simulink model "ZT_VehCtrl_18B_CAN"  (R2018b)
settings: Solver=FixedStepAuto  StartTime=0.0  StopTime=inf  FixedStep=0.005  RelTol=1e-3
InitFcn:
  | mbd_mpc_consistency_checks(bdroot(gcs));
values from neighbouring files (symbols this model uses):
  BatoverTempTh = single(80)    [VCU_INIT.m]
  BRS_PwrValid = single(5)    [VCU_INIT.m]
  BRSEnSpdTh1 = single(10)    [VCU_INIT.m]
  BRSEnSpdTh2 = single(20)    [VCU_INIT.m]
  MCUTempAlarmTh = single (60)    [VCU_INIT.m]
  mps2kmh = single(3.6)    [VCU_INIT.m]
  MtrPwrFac = single(1/9550)    [VCU_INIT.m]
  MtrTempAlarmTh = single (50)    [VCU_INIT.m]
  Padle1Signal1_Th = [PadleSignal1_min,PadleSignal1_max]    [VCU_INIT.m]
  Padle1Signal2_Th = [PadleSignal2_min,PadleSignal2_max]    [VCU_INIT.m]
  PadleSignal1_max = 3.84    [VCU_INIT.m]
  PadleSignal1_min = 0.75    [VCU_INIT.m]
  PadleSignal2_max = 1.92    [VCU_INIT.m]
  PadleSignal2_min = 0.375    [VCU_INIT.m]
  PadleValid = 0.05    [VCU_INIT.m]
  PwrLimFactor = single(0.5)    [VCU_INIT.m]
  Ratio = single(1)    [VCU_INIT.m]
  rpm2mps = single(2*pi/60 * WhlRadius/Ratio)    [VCU_INIT.m]
  SOCLowTh = single(20)    [VCU_INIT.m]
  VehPwrBackwardMax = VehPwrMax * single(0.3)    [VCU_INIT.m]
  VehPwrMax = single(MtrPwrMax * 4)    [VCU_INIT.m]
  VehTrqBackwardMax = VehTrqMax * single(0.3)    [VCU_INIT.m]
  VehTrqMax = single(MtrTrqMax * Ratio *4)    [VCU_INIT.m]
  WhlRadius = single(1)    [VCU_INIT.m]
undefined symbols (not defined in the file or in its folder): Delay_Charge, Delay_Discharge, fifo_0_vect, fifo_1_vect, LQFP, pts1_fifo_0_vect, pts1_fifo_1_vect, pts2_fifo_0_vect, pts2_fifo_1_vect, pts3_fifo_0_vect, pts3_fifo_1_vect, pts4_fifo_0_vect, pts4_fifo_1_vect
libraries: mbd_mpc574x_ec_toolbox x157, canmsglib x74, simulink x38
(part 9 of 12)

== system ZT_VehCtrl_18B_CAN/SigIn/CAN0 /BMS_Relay Status2/UNPACK ==
  ID : Inport
  data : Inport  Port=2
  length : Inport  Port=3
  timestamp : Inport  Port=4
  Action Port : ActionPort
  Bus Creator : BusCreator  Inputs=7  OutDataTypeStr=Bus: CAN_MESSAGE_BUS  NonVirtualBus=on
  Bus Creator1 : BusCreator  Inputs=2
  CAN Unpack6 : canmsglib/CAN Unpack  CANdbFile=D:\VCU\VCU_SL_ZhengZhou\ZT2\模型与接口\CAN_DBC\整车CANA_GBK.dbc  MsgList=(none)  MsgName=BMS_Relay_Status_2  MsgIDType=Standard (11-bit identifier)  MsgIdentifier=864  MsgLength=8  SignalInfo=NO1_RelayFaultStatus$9$2$2$2$1$0$1$0$0$3$#NO1_RelayIndex$11$5$2$2$1$0$1$0$0$31$#NO1_RelayStatus$8$1$2$2$1$0$1$0$0$1$#NO2_RelayFaultStatus$17$2$2$2$1$0$1$0$0$3$#NO2_RelayIndex$19$5$2$2$1$0$1$0$0$31$#NO2_RelayStatus$16$1$2$2$1$0$1$0$0$1$#NO3_RelayFaultStatus$25$2$2$2$1$0$1$0$0$3$#NO3_RelayIndex$27$5$2$2$1$0$1$0$0$31$#NO3_RelayStatus$24$1$2$2$1$0$1$0$0$1$#NO4_RelayFaultStatus$33$2$2$2$1$0$1$0$0$3$#NO4_RelayIndex$35$5$2$2$1$0$1$0$0$31$#NO4_RelayStatus$32$1$2$2$1$0$1$0$0$1$#NO5_RelayFaultStatus$41$2$2$2$1$0$1$0$0$3$#NO5_RelayIndex$43$5$2$2$1$0$1$0$0$31$#NO5_RelayStatus$40$1$2$2$1$0$1$0$0$1$#NO6_RelayFaultStatus$49$2$2$2$1$0$1$0$0$3$#NO6_RelayIndex$51$5$2$2$1$0$1$0$0$31$#NO6_RelayStatus$48$1$2$2$1$0$1$0$0$1$#NO7_RelayFaultStatus$57$2$2$2$1$0$1$0$0$3$#NO7_RelayIndex$59$5$2$2$1$0$1$0$0$31$#NO7_RelayStatus$56$1$2$2$1$0$1$0$0$1$#RelayNum$0$8$2$2$1$0$1$0$0$15$#  NSignals=22  IDPort=off  TimestampPort=off  ErrorPort=off  RemotePort=off  LengthPort=off  StatusPort=off  StartBits=str2num('[int32(9);int32(11);int32(8);int32(17);int32(19);int32(16);int32(25);int32(27);int32(24);int32(33);int32(35);int32(32);int32(41);int32(43);int32(40);int32(49);int32(51);int32(48);int32(57);int32(59);int32(56);int32(0)]')  SignalSizes=str2num('[int32(2);int32(5);int32(1);int32(2);int32(5);int32(1);int32(2);int32(5);int32(1);int32(2);int32(5);int32(1);int32(2);int32(5);int32(1);int32(2);int32(5);int32(1);int32(2);int32(5);int32(1);int32(8)]')  ByteOrders=str2num('[int32(2);int32(2);int32(2);int32(2);int32(2);int32(2);int32(2);int32(2);int32(2);int32(2);int32(2);int32(2);int32(2);int32(2);int32(2);int32(2);int32(2);int32(2);int32(2);int32(2);int32(2);int32(2)]')  DataTypes=str2num('[int32(2);int32(2);int32(2);int32(2);int32(2);int32(2);int32(2);int32(2);int32(2);int32(2);int32(2);int32(2);int32(2);int32(2);int32(2);int32(2);int32(2);int32(2);int32(2);int32(2);int32(2);int32(2)]')  MultiplexTypes=str2num('[int32(1);int32(1);int32(1);int32(1);int32(1);int32(1);int32(1);int32(1);int32(1);int32(1);int32(1);int32(1);int32(1);int32(1);int32(1);int32(1);int32(1);int32(1);int32(1);int32(1);int32(1);int32(1)]')  MultiplexValues=str2num('[double(0);double(0);double(0);double(0);double(0);double(0);double(0);double(0);double(0);double(0);double(0);double(0);double(0);double(0);double(0);double(0);double(0);double(0);double(0);double(0);double(0);double(0)]')  Factors=str2num('[double(1);double(1);double(1);double(1);double(1);double(1);double(1);double(1);double(1);double(1);double(1);double(1);double(1);double(1);double(1);double(1);double(1);double(1);double(1);double(1);double(1);double(1)]')  Offsets=str2num('[double(0);double(0);double(0);double(0);double(0);double(0);double(0);double(0);double(0);double(0);double(0);double(0);double(0);double(0);double(0);double(0);double(0);double(0);double(0);double(0);double(0);double(0)]')  Minimums=str2num('[double(0);double(0);double(0);double(0);double(0);double(0);double(0);double(0);double(0);double(0);double(0);double(0);double(0);double(0);double(0);double(0);double(0);double(0);double(0);double(0);double(0);double(0)]')  Maximums=str2num('[double(3);double(31);double(1);double(3);double(31);double(1);double(3);double(31);double(1);double(3);double(31);double(1);double(3);double(31);double(1);double(3);double(31);double(1);double(3);double(31);double(1);double(15)]')  ApplyMinMax=off
      settings: SourceProductName=Simulink Real-Time  SourceProductBaseCode=XP  DataFormat=CANdb specified signals
  Constant1 : Constant  Value=0  OutDataTypeStr=uint8
  Constant4 : Constant  Value=0  OutDataTypeStr=uint8
  Constant5 : Constant  Value=0  OutDataTypeStr=uint8
  Data Type Conversion{,14..15,17} (4 alike) : DataTypeConversion  OutDataTypeStr=uint8
  Data Type Conversion18 : DataTypeConversion  OutDataTypeStr=uint32
  Data Type Conversion19 : DataTypeConversion  OutDataTypeStr=double
  Message : Outport
  wires:
  Bus Creator1/1 -> Message/1
  Data Type Conversion15/1 -> Bus Creator/3  "Remote"
  Data Type Conversion14/1 -> Bus Creator/2  "Length"
  Data Type Conversion/1 -> Bus Creator/1  "Extended"
  Bus Creator/1 -> CAN Unpack6/1  "CAN_Msg_In"
  Data Type Conversion17/1 -> Bus Creator/4  "Error"
  timestamp/1 -> Data Type Conversion19/1
  Data Type Conversion19/1 -> Bus Creator/6  "Timestamp"
  ID/1 -> Data Type Conversion18/1
  Constant5/1 -> Data Type Conversion17/1
  Constant1/1 -> Data Type Conversion/1
  Data Type Conversion18/1 -> Bus Creator/5  "ID"
  data/1 -> Bus Creator/7  "Data"
  length/1 -> Data Type Conversion14/1
  Constant4/1 -> Data Type Conversion15/1

== system ZT_VehCtrl_18B_CAN/SigIn/CAN0 /BMS_Relay Status3/UNPACK ==
  ID : Inport
  data : Inport  Port=2
  length : Inport  Port=3
  timestamp : Inport  Port=4
  Action Port : ActionPort
  Bus Creator : BusCreator  Inputs=7  OutDataTypeStr=Bus: CAN_MESSAGE_BUS  NonVirtualBus=on
  Bus Creator1 : BusCreator  Inputs=2
  CAN Unpack6 : canmsglib/CAN Unpack  CANdbFile=D:\VCU\VCU_SL_ZhengZhou\ZT2\模型与接口\CAN_DBC\整车CANA_GBK.dbc  MsgList=(none)  MsgName=BMS_Relay_Status_3  MsgIDType=Standard (11-bit identifier)  MsgIdentifier=865  MsgLength=8  SignalInfo=NO10_RelayFaultStatus$17$2$2$2$1$0$1$0$0$1$#NO10_RelayIndex$19$5$2$2$1$0$1$0$0$1$#NO10_RelayStatus$16$1$2$2$1$0$1$0$0$1$#NO11_RelayFaultStatus$25$2$2$2$1$0$1$0$0$1$#NO11_RelayIndex$27$5$2$2$1$0$1$0$0$1$#NO11_RelayStatus$24$1$2$2$1$0$1$0$0$1$#NO12_RelayFaultStatus$33$2$2$2$1$0$1$0$0$1$#NO12_RelayIndex$35$5$2$2$1$0$1$0$0$1$#NO12_RelayStatus$32$1$2$2$1$0$1$0$0$1$#NO13_RelayFaultStatus$41$2$2$2$1$0$1$0$0$1$#NO13_RelayIndex$43$5$2$2$1$0$1$0$0$1$#NO13_RelayStatus$40$1$2$2$1$0$1$0$0$1$#NO14_RelayFaultStatus$49$2$2$2$1$0$1$0$0$1$#NO14_RelayIndex$51$5$2$2$1$0$1$0$0$1$#NO14_RelayStatus$48$1$2$2$1$0$1$0$0$1$#NO15_RelayFaultStatus$57$2$2$2$1$0$1$0$0$1$#NO15_RelayIndex$59$5$2$2$1$0$1$0$0$1$#NO15_RelayStatus$56$1$2$2$1$0$1$0$0$1$#NO8_RelayFaultStatus$1$2$2$2$1$0$1$0$0$1$#NO8_RelayIndex$3$5$2$2$1$0$1$0$0$1$#NO8_RelayStatus$0$1$2$2$1$0$1$0$0$1$#NO9_RelayFaultStatus$9$2$2$2$1$0$1$0$0$1$#NO9_RelayIndex$11$5$2$2$1$0$1$0$0$1$#NO9_RelayStatus$8$1$2$2$1$0$1$0$0$1$#  NSignals=24  IDPort=off  TimestampPort=off  ErrorPort=off  RemotePort=off  LengthPort=off  StatusPort=off  StartBits=str2num('[int32(17);int32(19);int32(16);int32(25);int32(27);int32(24);int32(33);int32(35);int32(32);int32(41);int32(43);int32(40);int32(49);int32(51);int32(48);int32(57);int32(59);int32(56);int32(1);int32(3);int32(0);int32(9);int32(11);int32(8)]')  SignalSizes=str2num('[int32(2);int32(5);int32(1);int32(2);int32(5);int32(1);int32(2);int32(5);int32(1);int32(2);int32(5);int32(1);int32(2);int32(5);int32(1);int32(2);int32(5);int32(1);int32(2);int32(5);int32(1);int32(2);int32(5);int32(1)]')  ByteOrders=str2num('[int32(2);int32(2);int32(2);int32(2);int32(2);int32(2);int32(2);int32(2);int32(2);int32(2);int32(2);int32(2);int32(2);int32(2);int32(2);int32(2);int32(2);int32(2);int32(2);int32(2);int32(2);int32(2);int32(2);int32(2)]')  DataTypes=str2num('[int32(2);int32(2);int32(2);int32(2);int32(2);int32(2);int32(2);int32(2);int32(2);int32(2);int32(2);int32(2);int32(2);int32(2);int32(2);int32(2);int32(2);int32(2);int32(2);int32(2);int32(2);int32(2);int32(2);int32(2)]')  MultiplexTypes=str2num('[int32(1);int32(1);int32(1);int32(1);int32(1);int32(1);int32(1);int32(1);int32(1);int32(1);int32(1);int32(1);int32(1);int32(1);int32(1);int32(1);int32(1);int32(1);int32(1);int32(1);int32(1);int32(1);int32(1);int32(1)]')  MultiplexValues=str2num('[double(0);double(0);double(0);double(0);double(0);double(0);double(0);double(0);double(0);double(0);double(0);double(0);double(0);double(0);double(0);double(0);double(0);double(0);double(0);double(0);double(0);double(0);double(0);double(0)]')  Factors=str2num('[double(1);double(1);double(1);double(1);double(1);double(1);double(1);double(1);double(1);double(1);double(1);double(1);double(1);double(1);double(1);double(1);double(1);double(1);double(1);double(1);double(1);double(1);double(1);double(1)]')  Offsets=str2num('[double(0);double(0);double(0);double(0);double(0);double(0);double(0);double(0);double(0);double(0);double(0);double(0);double(0);double(0);double(0);double(0);double(0);double(0);double(0);double(0);double(0);double(0);double(0);double(0)]')  Minimums=str2num('[double(0);double(0);double(0);double(0);double(0);double(0);double(0);double(0);double(0);double(0);double(0);double(0);double(0);double(0);double(0);double(0);double(0);double(0);double(0);double(0);double(0);double(0);double(0);double(0)]')  Maximums=str2num('[double(1);double(1);double(1);double(1);double(1);double(1);double(1);double(1);double(1);double(1);double(1);double(1);double(1);double(1);double(1);double(1);double(1);double(1);double(1);double(1);double(1);double(1);double(1);double(1)]')  ApplyMinMax=off
      settings: SourceProductName=Simulink Real-Time  SourceProductBaseCode=XP  DataFormat=CANdb specified signals
  Constant1 : Constant  Value=0  OutDataTypeStr=uint8
  Constant4 : Constant  Value=0  OutDataTypeStr=uint8
  Constant5 : Constant  Value=0  OutDataTypeStr=uint8
  Data Type Conversion{,14..15,17} (4 alike) : DataTypeConversion  OutDataTypeStr=uint8
  Data Type Conversion18 : DataTypeConversion  OutDataTypeStr=uint32
  Data Type Conversion19 : DataTypeConversion  OutDataTypeStr=double
  Message : Outport
  wires:
  Constant4/1 -> Data Type Conversion15/1
  length/1 -> Data Type Conversion14/1
  data/1 -> Bus Creator/7  "Data"
  Data Type Conversion18/1 -> Bus Creator/5  "ID"
  Constant1/1 -> Data Type Conversion/1
  Constant5/1 -> Data Type Conversion17/1
  ID/1 -> Data Type Conversion18/1
  Data Type Conversion19/1 -> Bus Creator/6  "Timestamp"
  timestamp/1 -> Data Type Conversion19/1
  Data Type Conversion17/1 -> Bus Creator/4  "Error"
  Bus Creator/1 -> CAN Unpack6/1  "CAN_Msg_In"
  Data Type Conversion/1 -> Bus Creator/1  "Extended"
  Data Type Conversion14/1 -> Bus Creator/2  "Length"
  Data Type Conversion15/1 -> Bus Creator/3  "Remote"
  Bus Creator1/1 -> Message/1

== system ZT_VehCtrl_18B_CAN/SigIn/CAN0 /BRS2VCU1/UNPACK ==
  ID : Inport
  data : Inport  Port=2
  length : Inport  Port=3
  timestamp : Inport  Port=4
  Action Port : ActionPort  ActionType=case
  Add : Sum
  Bus Creator : BusCreator  Inputs=7  OutDataTypeStr=Bus: CAN_MESSAGE_BUS  NonVirtualBus=on
  Bus Creator1 : BusCreator  Inputs=5
  CAN Unpack6 : canmsglib/CAN Unpack  CANdbFile=D:\VCU\VCU_SL_ZhengZhou\ZT2\模型与接口\CAN_DBC\整车CANA_GBK.dbc  MsgList=(none)  MsgName=BRS2VCU1  MsgIDType=Extended (29-bit identifier)  MsgIdentifier=419309028  MsgLength=8  SignalInfo=ActualPower$16$16$1$2$1$0$1$0$0$500$#BrakeResistorTemp$32$16$1$2$1$0$1$-40$-40$470$#ControllerTemp$48$8$1$2$1$0$1$-40$-40$470$#FaultLevel$14$2$1$2$1$0$1$0$0$3$#OperationMode$4$4$1$2$1$0$1$0$0$15$#  NSignals=5  IDPort=off  TimestampPort=off  ErrorPort=off  RemotePort=off  LengthPort=off  StatusPort=off  StartBits=str2num('[int32(16);int32(32);int32(48);int32(14);int32(4)]')  SignalSizes=str2num('[int32(16);int32(16);int32(8);int32(2);int32(4)]')  ByteOrders=str2num('[int32(1);int32(1);int32(1);int32(1);int32(1)]')  DataTypes=str2num('[int32(2);int32(2);int32(2);int32(2);int32(2)]')  MultiplexTypes=str2num('[int32(1);int32(1);int32(1);int32(1);int32(1)]')  MultiplexValues=str2num('[double(0);double(0);double(0);double(0);double(0)]')  Factors=str2num('[double(1);double(1);double(1);double(1);double(1)]')  Offsets=str2num('[double(0);double(-40);double(-40);double(0);double(0)]')  Minimums=str2num('[double(0);double(-40);double(-40);double(0);double(0)]')  Maximums=str2num('[double(500);double(470);double(470);double(3);double(15)]')  ApplyMinMax=off
      settings: SourceProductName=Simulink Real-Time  SourceProductBaseCode=XP  DataFormat=CANdb specified signals
  Constant : Constant  OutDataTypeStr=uint8
  Constant1 : Constant  OutDataTypeStr=uint8
  Constant4 : Constant  Value=0  OutDataTypeStr=uint8
  Constant5 : Constant  Value=0  OutDataTypeStr=uint8
  Data Store Read : DataStoreRead  DataStoreName=Cnt_BRS1
  Data Store Write : DataStoreWrite  DataStoreName=Cnt_BRS1
  Data Type Conversion{,14..15,17} (4 alike) : DataTypeConversion  OutDataTypeStr=uint8
  Data Type Conversion{1..5} (5 alike) : DataTypeConversion  OutDataTypeStr=single
  Data Type Conversion18 : DataTypeConversion  OutDataTypeStr=uint32
  Data Type Conversion19 : DataTypeConversion  OutDataTypeStr=double
  Message : Outport
  wires:
  Constant4/1 -> Data Type Conversion15/1
  length/1 -> Data Type Conversion14/1
  data/1 -> Bus Creator/7  "Data"
  Data Type Conversion18/1 -> Bus Creator/5  "ID"
  Constant1/1 -> Data Type Conversion/1
  Constant5/1 -> Data Type Conversion17/1
  ID/1 -> Data Type Conversion18/1
  Data Type Conversion19/1 -> Bus Creator/6  "Timestamp"
  timestamp/1 -> Data Type Conversion19/1
  Data Type Conversion17/1 -> Bus Creator/4  "Error"
  Bus Creator/1 -> CAN Unpack6/1  "CAN_Msg_In"
  Data Type Conversion/1 -> Bus Creator/1  "Extended"
  Data Type Conversion14/1 -> Bus Creator/2  "Length"
  Data Type Conversion15/1 -> Bus Creator/3  "Remote"
  Bus Creator1/1 -> Message/1
  CAN Unpack6/1 -> Data Type Conversion5/1
  CAN Unpack6/2 -> Data Type Conversion4/1
  CAN Unpack6/3 -> Data Type Conversion3/1
  CAN Unpack6/4 -> Data Type Conversion2/1
  CAN Unpack6/5 -> Data Type Conversion1/1
  Data Type Conversion1/1 -> Bus Creator1/5  "OperationMode"
  Data Type Conversion2/1 -> Bus Creator1/4  "FaultLevel"
  Data Type Conversion3/1 -> Bus Creator1/3  "ControllerTemp"
  Data Type Conversion4/1 -> Bus Creator1/2  "BrakeResistorTemp"
  Data Type Conversion5/1 -> Bus Creator1/1  "ActualPower"
  Constant/1 -> Add/2
  Data Store Read/1 -> Add/1
  Add/1 -> Data Store Write/1

== system ZT_VehCtrl_18B_CAN/SigIn/CAN0 /BRS2VCU2/UNPACK ==
  ID : Inport
  data : Inport  Port=2
  length : Inport  Port=3
  timestamp : Inport  Port=4
  Action Port : ActionPort  ActionType=case
  Add : Sum
  Bus Creator : BusCreator  Inputs=7  OutDataTypeStr=Bus: CAN_MESSAGE_BUS  NonVirtualBus=on
  Bus Creator1 : BusCreator  Inputs=4
  CAN Unpack6 : canmsglib/CAN Unpack  CANdbFile=D:\VCU\VCU_SL_ZhengZhou\ZT2\模型与接口\CAN_DBC\整车CANA_GBK.dbc  MsgList=(none)  MsgName=BRS2VCU2  MsgIDType=Extended (29-bit identifier)  MsgIdentifier=419309284  MsgLength=8  SignalInfo=AvailableMaxPower$32$16$1$2$1$0$1$0$0$500$#BusVoltageMeasured$48$16$1$2$1$0$1.000000e-01$0$0$1000$#BusVoltageReceived$0$16$1$2$1$0$1$0$0$1000$#OperatingCurrent$16$16$1$2$1$0$1$0$0$1000$#  NSignals=4  IDPort=off  TimestampPort=off  ErrorPort=off  RemotePort=off  LengthPort=off  StatusPort=off  StartBits=str2num('[int32(32);int32(48);int32(0);int32(16)]')  SignalSizes=str2num('[int32(16);int32(16);int32(16);int32(16)]')  ByteOrders=str2num('[int32(1);int32(1);int32(1);int32(1)]')  DataTypes=str2num('[int32(2);int32(2);int32(2);int32(2)]')  MultiplexTypes=str2num('[int32(1);int32(1);int32(1);int32(1)]')  MultiplexValues=str2num('[double(0);double(0);double(0);double(0)]')  Factors=str2num('[double(1);double(1.000000e-01);double(1);double(1)]')  Offsets=str2num('[double(0);double(0);double(0);double(0)]')  Minimums=str2num('[double(0);double(0);double(0);double(0)]')  Maximums=str2num('[double(500);double(1000);double(1000);double(1000)]')  ApplyMinMax=off
      settings: SourceProductName=Simulink Real-Time  SourceProductBaseCode=XP  DataFormat=CANdb specified signals
  Constant : Constant  OutDataTypeStr=uint8
  Constant1 : Constant  OutDataTypeStr=uint8
  Constant4 : Constant  Value=0  OutDataTypeStr=uint8
  Constant5 : Constant  Value=0  OutDataTypeStr=uint8
  Data Store Read : DataStoreRead  DataStoreName=Cnt_BRS2
  Data Store Write : DataStoreWrite  DataStoreName=Cnt_BRS2
  Data Type Conversion{,14..15,17} (4 alike) : DataTypeConversion  OutDataTypeStr=uint8
  Data Type Conversion{1..4} (4 alike) : DataTypeConversion  OutDataTypeStr=single
  Data Type Conversion18 : DataTypeConversion  OutDataTypeStr=uint32
  Data Type Conversion19 : DataTypeConversion  OutDataTypeStr=double
  Message : Outport
  wires:
  Bus Creator1/1 -> Message/1
  Data Type Conversion15/1 -> Bus Creator/3  "Remote"
  Data Type Conversion14/1 -> Bus Creator/2  "Length"
  Data Type Conversion/1 -> Bus Creator/1  "Extended"
  Bus Creator/1 -> CAN Unpack6/1  "CAN_Msg_In"
  Data Type Conversion17/1 -> Bus Creator/4  "Error"
  timestamp/1 -> Data Type Conversion19/1
  Data Type Conversion19/1 -> Bus Creator/6  "Timestamp"
  ID/1 -> Data Type Conversion18/1
  Constant5/1 -> Data Type Conversion17/1
  Constant1/1 -> Data Type Conversion/1
  Data Type Conversion18/1 -> Bus Creator/5  "ID"
  data/1 -> Bus Creator/7  "Data"
  length/1 -> Data Type Conversion14/1
  Constant4/1 -> Data Type Conversion15/1
  CAN Unpack6/1 -> Data Type Conversion4/1
  CAN Unpack6/2 -> Data Type Conversion3/1
  CAN Unpack6/3 -> Data Type Conversion2/1
  CAN Unpack6/4 -> Data Type Conversion1/1
  Data Type Conversion1/1 -> Bus Creator1/4  "OperatingCurrent"
  Data Type Conversion2/1 -> Bus Creator1/3  "BusVoltageReceived"
  Data Type Conversion3/1 -> Bus Creator1/2  "BusVoltageMeasured"
  Data Type Conversion4/1 -> Bus Creator1/1  "AvailableMaxPower"
  Add/1 -> Data Store Write/1
  Constant/1 -> Add/2
  Data Store Read/1 -> Add/1

== system ZT_VehCtrl_18B_CAN/SigIn/CAN0 /BRS2VCU3/UNPACK ==
  ID : Inport
  data : Inport  Port=2
  length : Inport  Port=3
  timestamp : Inport  Port=4
  Action Port : ActionPort  ActionType=case
  Add : Sum
  Bus Creator : BusCreator  Inputs=7  OutDataTypeStr=Bus: CAN_MESSAGE_BUS  NonVirtualBus=on
  Bus Creator1 : BusCreator  Inputs=3
  CAN Unpack6 : canmsglib/CAN Unpack  CANdbFile=D:\VCU\VCU_SL_ZhengZhou\ZT2\模型与接口\CAN_DBC\整车CANA_GBK.dbc  MsgList=(none)  MsgName=BRS2VCU3  MsgIDType=Extended (29-bit identifier)  MsgIdentifier=419309540  MsgLength=8  SignalInfo=DutyCycle$0$8$1$2$1$0$1$0$0$100$#EnvironmentTemp$16$16$1$2$1$0$1$-40$-40$470$#FanTemp$32$16$1$2$1$0$1$-40$-40$470$#  NSignals=3  IDPort=off  TimestampPort=off  ErrorPort=off  RemotePort=off  LengthPort=off  StatusPort=off  StartBits=str2num('[int32(0);int32(16);int32(32)]')  SignalSizes=str2num('[int32(8);int32(16);int32(16)]')  ByteOrders=str2num('[int32(1);int32(1);int32(1)]')  DataTypes=str2num('[int32(2);int32(2);int32(2)]')  MultiplexTypes=str2num('[int32(1);int32(1);int32(1)]')  MultiplexValues=str2num('[double(0);double(0);double(0)]')  Factors=str2num('[double(1);double(1);double(1)]')  Offsets=str2num('[double(0);double(-40);double(-40)]')  Minimums=str2num('[double(0);double(-40);double(-40)]')  Maximums=str2num('[double(100);double(470);double(470)]')  ApplyMinMax=off
      settings: SourceProductName=Simulink Real-Time  SourceProductBaseCode=XP  DataFormat=CANdb specified signals
  Constant : Constant  OutDataTypeStr=uint8
  Constant1 : Constant  OutDataTypeStr=uint8
  Constant4 : Constant  Value=0  OutDataTypeStr=uint8
  Constant5 : Constant  Value=0  OutDataTypeStr=uint8
  Data Store Read : DataStoreRead  DataStoreName=Cnt_BRS3
  Data Store Write : DataStoreWrite  DataStoreName=Cnt_BRS3
  Data Type Conversion{,14..15,17} (4 alike) : DataTypeConversion  OutDataTypeStr=uint8
  Data Type Conversion1 : DataTypeConversion  OutDataTypeStr=single
  Data Type Conversion18 : DataTypeConversion  OutDataTypeStr=uint32
  Data Type Conversion19 : DataTypeConversion  OutDataTypeStr=double
  Data Type Conversion2 : DataTypeConversion  OutDataTypeStr=single
  Data Type Conversion3 : DataTypeConversion  OutDataTypeStr=single
  Message : Outport
  wires:
  Constant4/1 -> Data Type Conversion15/1
  length/1 -> Data Type Conversion14/1
  data/1 -> Bus Creator/7  "Data"
  Data Type Conversion18/1 -> Bus Creator/5  "ID"
  Constant1/1 -> Data Type Conversion/1
  Constant5/1 -> Data Type Conversion17/1
  ID/1 -> Data Type Conversion18/1
  Data Type Conversion19/1 -> Bus Creator/6  "Timestamp"
  timestamp/1 -> Data Type Conversion19/1
  Data Type Conversion17/1 -> Bus Creator/4  "Error"
  Bus Creator/1 -> CAN Unpack6/1  "CAN_Msg_In"
  Data Type Conversion/1 -> Bus Creator/1  "Extended"
  Data Type Conversion14/1 -> Bus Creator/2  "Length"
  Data Type Conversion15/1 -> Bus Creator/3  "Remote"
  Bus Creator1/1 -> Message/1
  CAN Unpack6/1 -> Data Type Conversion1/1
  CAN Unpack6/2 -> Data Type Conversion2/1
  CAN Unpack6/3 -> Data Type Conversion3/1
  Data Type Conversion1/1 -> Bus Creator1/1  "DutyCycle"
  Data Type Conversion2/1 -> Bus Creator1/2  "EnvironmentTemp"
  Data Type Conversion3/1 -> Bus Creator1/3  "FanTemp"
  Data Store Read/1 -> Add/1
  Constant/1 -> Add/2
  Add/1 -> Data Store Write/1

== system ZT_VehCtrl_18B_CAN/SigIn/CAN0 /OBC_Charger Status/UNPACK ==
  ID : Inport
  data : Inport  Port=2
  length : Inport  Port=3
  timestamp : Inport  Port=4
  Action Port : ActionPort  ActionType=case
  Add : Sum
  Bus Creator : BusCreator  Inputs=7  OutDataTypeStr=Bus: CAN_MESSAGE_BUS  NonVirtualBus=on
  Bus Creator1 : BusCreator  Inputs=8
  CAN Unpack6 : canmsglib/CAN Unpack  CANdbFile=D:\VCU\VCU_SL_ZhengZhou\ZT2\模型与接口\CAN_DBC\整车CANA_GBK.dbc  MsgList=(none)  MsgName=OBC_Charger_Status  MsgIDType=Standard (11-bit identifier)  MsgIdentifier=544  MsgLength=8  SignalInfo=OBC_ComSt$36$1$2$2$1$0$1$0$0$1$#OBC_Current$24$16$2$2$1$0$1.000000e-01$0$0$1000$#OBC_HwFault$32$1$2$2$1$0$1$0$0$1$#OBC_InputVoltage$34$1$2$2$1$0$1$0$0$1$#OBC_OutputShortCircuit$37$1$2$2$1$0$1$0$0$1$#OBC_StartSt$35$1$2$2$1$0$1$0$0$1$#OBC_Temp$33$1$2$2$1$0$1$0$0$1$#OBC_Voltage$8$16$2$2$1$0$1.000000e-01$0$0$1000$#  NSignals=8  IDPort=off  TimestampPort=off  ErrorPort=off  RemotePort=off  LengthPort=off  StatusPort=off  StartBits=str2num('[int32(36);int32(24);int32(32);int32(34);int32(37);int32(35);int32(33);int32(8)]')  SignalSizes=str2num('[int32(1);int32(16);int32(1);int32(1);int32(1);int32(1);int32(1);int32(16)]')  ByteOrders=str2num('[int32(2);int32(2);int32(2);int32(2);int32(2);int32(2);int32(2);int32(2)]')  DataTypes=str2num('[int32(2);int32(2);int32(2);int32(2);int32(2);int32(2);int32(2);int32(2)]')  MultiplexTypes=str2num('[int32(1);int32(1);int32(1);int32(1);int32(1);int32(1);int32(1);int32(1)]')  MultiplexValues=str2num('[double(0);double(0);double(0);double(0);double(0);double(0);double(0);double(0)]')  Factors=str2num('[double(1);double(1.000000e-01);double(1);double(1);double(1);double(1);double(1);double(1.000000e-01)]')  Offsets=str2num('[double(0);double(0);double(0);double(0);double(0);double(0);double(0);double(0)]')  Minimums=str2num('[double(0);double(0);double(0);double(0);double(0);double(0);double(0);double(0)]')  Maximums=str2num('[double(1);double(1000);double(1);double(1);double(1);double(1);double(1);double(1000)]')  ApplyMinMax=off
      settings: SourceProductName=Simulink Real-Time  SourceProductBaseCode=XP  DataFormat=CANdb specified signals
  Constant : Constant  OutDataTypeStr=uint8
  Constant1 : Constant  Value=0  OutDataTypeStr=uint8
  Constant4 : Constant  Value=0  OutDataTypeStr=uint8
  Constant5 : Constant  Value=0  OutDataTypeStr=uint8
  Data Store Read : DataStoreRead  DataStoreName=Cnt_OBC
  Data Store Write : DataStoreWrite  DataStoreName=Cnt_OBC
  Data Type Conversion{,14..15,17} (4 alike) : DataTypeConversion  OutDataTypeStr=uint8
  Data Type Conversion{1,3..7} (6 alike) : DataTypeConversion  OutDataTypeStr=boolean
  Data Type Conversion18 : DataTypeConversion  OutDataTypeStr=uint32
  Data Type Conversion19 : DataTypeConversion  OutDataTypeStr=double
  Data Type Conversion2 : DataTypeConversion  OutDataTypeStr=single
  Data Type Conversion8 : DataTypeConversion  OutDataTypeStr=single
  Message : Outport
  wires:
  Constant4/1 -> Data Type Conversion15/1
  length/1 -> Data Type Conversion14/1
  data/1 -> Bus Creator/7  "Data"
  Data Type Conversion18/1 -> Bus Creator/5  "ID"
  Constant1/1 -> Data Type Conversion/1
  Constant5/1 -> Data Type Conversion17/1
  ID/1 -> Data Type Conversion18/1
  Data Type Conversion19/1 -> Bus Creator/6  "Timestamp"
  timestamp/1 -> Data Type Conversion19/1
  Data Type Conversion17/1 -> Bus Creator/4  "Error"
  Bus Creator/1 -> CAN Unpack6/1  "CAN_Msg_In"
  Data Type Conversion/1 -> Bus Creator/1  "Extended"
  Data Type Conversion14/1 -> Bus Creator/2  "Length"
  Data Type Conversion15/1 -> Bus Creator/3  "Remote"
  Bus Creator1/1 -> Message/1
  CAN Unpack6/1 -> Data Type Conversion1/1
  CAN Unpack6/2 -> Data Type Conversion2/1
  CAN Unpack6/3 -> Data Type Conversion3/1
  CAN Unpack6/4 -> Data Type Conversion4/1
  CAN Unpack6/5 -> Data Type Conversion5/1
  CAN Unpack6/6 -> Data Type Conversion6/1
  CAN Unpack6/7 -> Data Type Conversion7/1
  CAN Unpack6/8 -> Data Type Conversion8/1
  Data Type Conversion1/1 -> Bus Creator1/1  "OBC_ComSt"
  Data Type Conversion2/1 -> Bus Creator1/2  "OBC_Current"
  Data Type Conversion3/1 -> Bus Creator1/3  "OBC_HwFault"
  Data Type Conversion4/1 -> Bus Creator1/4  "OBC_InputVoltage"
  Data Type Conversion5/1 -> Bus Creator1/5  "OBC_OutputShortCircuit"
  Data Type Conversion6/1 -> Bus Creator1/6  "OBC_StartSt"
  Data Type Conversion7/1 -> Bus Creator1/7  "OBC_Temp"
  Data Type Conversion8/1 -> Bus Creator1/8  "OBC_Voltage"
  Constant/1 -> Add/2
  Data Store Read/1 -> Add/1
  Add/1 -> Data Store Write/1

== system ZT_VehCtrl_18B_CAN/SigIn/CAN0 /PDU_RelaySts/UNPACK ==
  ID : Inport
  data : Inport  Port=2
  length : Inport  Port=3
  timestamp : Inport  Port=4
  Action Port : ActionPort
  Add : Sum
  Bus Creator : BusCreator  Inputs=7  OutDataTypeStr=Bus: CAN_MESSAGE_BUS  NonVirtualBus=on
  Bus Creator1 : BusCreator  Inputs=7
  CAN Unpack6 : canmsglib/CAN Unpack  CANdbFile=D:\VCU\VCU_SL_ZhengZhou\ZT2\模型与接口\CAN_DBC\动力CANB_GBK.dbc  MsgList=(none)  MsgName=PDU_RelaySts  MsgIDType=Extended (29-bit identifier)  MsgIdentifier=419376072  MsgLength=8  SignalInfo=MultiOne_HVACPcgRlySts$10$2$1$2$1$0$1$0$-Inf$Inf$#PDU_HVACRlySts$6$2$1$2$1$0$1$0$-Inf$Inf$#PDU_HrtBt$56$8$1$2$1$0$1$0$-Inf$Inf$#PDU_PTCRlySts$8$2$1$2$1$0$1$0$-Inf$Inf$#PDU_PosRlyPcgRlySts$4$2$1$2$1$0$1$0$-Inf$Inf$#PDU_PosRlySts$2$2$1$2$1$0$1$0$-Inf$Inf$#PDU_ShrRlySts$0$2$1$2$1$0$1$0$-Inf$Inf$#  NSignals=7  IDPort=off  TimestampPort=off  ErrorPort=off  RemotePort=off  LengthPort=off  StatusPort=off  StartBits=str2num('[int32(10);int32(6);int32(56);int32(8);int32(4);int32(2);int32(0)]')  SignalSizes=str2num('[int32(2);int32(2);int32(8);int32(2);int32(2);int32(2);int32(2)]')  ByteOrders=str2num('[int32(1);int32(1);int32(1);int32(1);int32(1);int32(1);int32(1)]')  DataTypes=str2num('[int32(2);int32(2);int32(2);int32(2);int32(2);int32(2);int32(2)]')  MultiplexTypes=str2num('[int32(1);int32(1);int32(1);int32(1);int32(1);int32(1);int32(1)]')  MultiplexValues=str2num('[double(0);double(0);double(0);double(0);double(0);double(0);double(0)]')  Factors=str2num('[double(1);double(1);double(1);double(1);double(1);double(1);double(1)]')  Offsets=str2num('[double(0);double(0);double(0);double(0);double(0);double(0);double(0)]')  Minimums=str2num('[double(-Inf);double(-Inf);double(-Inf);double(-Inf);double(-Inf);double(-Inf);double(-Inf)]')  Maximums=str2num('[double(Inf);double(Inf);double(Inf);double(Inf);double(Inf);double(Inf);double(Inf)]')  ApplyMinMax=off
      settings: SourceProductName=Simulink Real-Time  SourceProductBaseCode=XP  DataFormat=CANdb specified signals
  Constant : Constant  OutDataTypeStr=uint8
  Constant1 : Constant  OutDataTypeStr=uint8
  Constant4 : Constant  Value=0  OutDataTypeStr=uint8
  Constant5 : Constant  Value=0  OutDataTypeStr=uint8
  Data Store Read : DataStoreRead  DataStoreName=Cnt_PDU
  Data Store Write : DataStoreWrite  DataStoreName=Cnt_PDU
  Data Type Conversion{,14..15,17} (4 alike) : DataTypeConversion  OutDataTypeStr=uint8
  Data Type Conversion{1..7} (7 alike) : DataTypeConversion  OutDataTypeStr=single
  Data Type Conversion18 : DataTypeConversion  OutDataTypeStr=uint32
  Data Type Conversion19 : DataTypeConversion  OutDataTypeStr=double
  Message : Outport
  wires:
  Bus Creator1/1 -> Message/1
  Data Type Conversion15/1 -> Bus Creator/3  "Remote"
  Data Type Conversion14/1 -> Bus Creator/2  "Length"
  Data Type Conversion/1 -> Bus Creator/1  "Extended"
  Bus Creator/1 -> CAN Unpack6/1  "CAN_Msg_In"
  Data Type Conversion17/1 -> Bus Creator/4  "Error"
  timestamp/1 -> Data Type Conversion19/1
  Data Type Conversion19/1 -> Bus Creator/6  "Timestamp"
  ID/1 -> Data Type Conversion18/1
  Constant5/1 -> Data Type Conversion17/1
  Constant1/1 -> Data Type Conversion/1
  Data Type Conversion18/1 -> Bus Creator/5  "ID"
  data/1 -> Bus Creator/7  "Data"
  length/1 -> Data Type Conversion14/1
  Constant4/1 -> Data Type Conversion15/1
  CAN Unpack6/1 -> Data Type Conversion1/1
  CAN Unpack6/2 -> Data Type Conversion2/1
  CAN Unpack6/3 -> Data Type Conversion3/1
  CAN Unpack6/4 -> Data Type Conversion4/1
  CAN Unpack6/5 -> Data Type Conversion5/1
  CAN Unpack6/6 -> Data Type Conversion6/1
  CAN Unpack6/7 -> Data Type Conversion7/1
  Data Type Conversion1/1 -> Bus Creator1/1  "MultiOne_HVACPcgRlySts"
  Data Type Conversion2/1 -> Bus Creator1/2  "PDU_HVACRlySts"
  Data Type Conversion3/1 -> Bus Creator1/3  "PDU_HrtBt"
  Data Type Conversion4/1 -> Bus Creator1/4  "PDU_PTCRlySts"
  Data Type Conversion5/1 -> Bus Creator1/5  "PDU_PosRlyPcgRlySts"
  Data Type Conversion6/1 -> Bus Creator1/6  "PDU_PosRlySts"
  Data Type Conversion7/1 -> Bus Creator1/7  "PDU_ShrRlySts"
  Constant/1 -> Add/2
  Data Store Read/1 -> Add/1
  Add/1 -> Data Store Write/1

== system ZT_VehCtrl_18B_CAN/SigIn/CAN0 /TMS2VCU/UNPACK ==
  ID : Inport
  data : Inport  Port=2
  length : Inport  Port=3
  timestamp : Inport  Port=4
  Action Port : ActionPort  ActionType=case
  Add : Sum
  Bus Creator : BusCreator  Inputs=7  OutDataTypeStr=Bus: CAN_MESSAGE_BUS  NonVirtualBus=on
  Bus Creator1 : BusCreator  Inputs=2
  CAN Unpack6 : canmsglib/CAN Unpack  CANdbFile=D:\VCU\VCU_SL_ZhengZhou\ZT2\模型与接口\CAN_DBC\整车CANA_GBK.dbc  MsgList=(none)  MsgName=TMS2VCU  MsgIDType=Extended (29-bit identifier)  MsgIdentifier=419427142  MsgLength=8  SignalInfo=TMS_FanSpeedLvl_num$0$8$2$2$1$0$1$0$0$255$#TMS_Life1_num$56$8$2$2$1$0$1$0$0$255$#  NSignals=2  IDPort=off  TimestampPort=off  ErrorPort=off  RemotePort=off  LengthPort=off  StatusPort=off  StartBits=str2num('[int32(0);int32(56)]')  SignalSizes=str2num('[int32(8);int32(8)]')  ByteOrders=str2num('[int32(2);int32(2)]')  DataTypes=str2num('[int32(2);int32(2)]')  MultiplexTypes=str2num('[int32(1);int32(1)]')  MultiplexValues=str2num('[double(0);double(0)]')  Factors=str2num('[double(1);double(1)]')  Offsets=str2num('[double(0);double(0)]')  Minimums=str2num('[double(0);double(0)]')  Maximums=str2num('[double(255);double(255)]')  ApplyMinMax=off
      settings: SourceProductName=Simulink Real-Time  SourceProductBaseCode=XP  DataFormat=CANdb specified signals
  Constant : Constant  OutDataTypeStr=uint8
  Constant1 : Constant  Value=0  OutDataTypeStr=uint8
  Constant4 : Constant  Value=0  OutDataTypeStr=uint8
  Constant5 : Constant  Value=0  OutDataTypeStr=uint8
  Data Store Read : DataStoreRead  DataStoreName=Cnt_TMS
  Data Store Write : DataStoreWrite  DataStoreName=Cnt_TMS
  Data Type Conversion{,14..15,17} (4 alike) : DataTypeConversion  OutDataTypeStr=uint8
  Data Type Conversion1 : DataTypeConversion  OutDataTypeStr=single
  Data Type Conversion18 : DataTypeConversion  OutDataTypeStr=uint32
  Data Type Conversion19 : DataTypeConversion  OutDataTypeStr=double
  Data Type Conversion2 : DataTypeConversion  OutDataTypeStr=single
  Message : Outport
  wires:
  Bus Creator1/1 -> Message/1
  Data Type Conversion15/1 -> Bus Creator/3  "Remote"
  Data Type Conversion14/1 -> Bus Creator/2  "Length"
  Data Type Conversion/1 -> Bus Creator/1  "Extended"
  Bus Creator/1 -> CAN Unpack6/1  "CAN_Msg_In"
  Data Type Conversion17/1 -> Bus Creator/4  "Error"
  timestamp/1 -> Data Type Conversion19/1
  Data Type Conversion19/1 -> Bus Creator/6  "Timestamp"
  ID/1 -> Data Type Conversion18/1
  Constant5/1 -> Data Type Conversion17/1
  Constant1/1 -> Data Type Conversion/1
  Data Type Conversion18/1 -> Bus Creator/5  "ID"
  data/1 -> Bus Creator/7  "Data"
  length/1 -> Data Type Conversion14/1
  Constant4/1 -> Data Type Conversion15/1
  CAN Unpack6/1 -> Data Type Conversion1/1
  CAN Unpack6/2 -> Data Type Conversion2/1
  Data Type Conversion1/1 -> Bus Creator1/1  "TMS_FanSpeedLvl_num"
  Data Type Conversion2/1 -> Bus Creator1/2  "TMS_Life1_num"
  Constant/1 -> Add/2
  Data Store Read/1 -> Add/1
  Add/1 -> Data Store Write/1

== system ZT_VehCtrl_18B_CAN/SigIn/CAN1/DCDC1_1/UNPACK ==
  ID : Inport
  data : Inport  Port=2
  length : Inport  Port=3
  timestamp : Inport  Port=4
  Action Port : ActionPort  ActionType=case
  Add : Sum
  Bus Creator : BusCreator  Inputs=7  OutDataTypeStr=Bus: CAN_MESSAGE_BUS  NonVirtualBus=on
  Bus Creator1 : BusCreator  Inputs=4
  CAN Unpack6 : canmsglib/CAN Unpack  CANdbFile=D:\VCU\VCU_SL_ZhengZhou\ZT2\Module\CAN_DBC\动力CANB_GBK.dbc  MsgList=(none)  MsgName=DCDC1_1  MsgIDType=Extended (29-bit identifier)  MsgIdentifier=402706575  MsgLength=8  SignalInfo=DCDC1_InputVolt$32$16$1$2$1$0$1.000000e-01$0$0$1000$#DCDC1_ModuleTemp$48$8$1$2$1$0$1$-40$-40$215$#DCDC1_OutCurr$16$16$1$2$1$0$1.000000e-01$0$0$1000$#DCDC1_OutVolt$0$16$1$2$1$0$1.000000e-01$0$0$1000$#  NSignals=4  IDPort=off  TimestampPort=off  ErrorPort=off  RemotePort=off  LengthPort=off  StatusPort=off  StartBits=str2num('[int32(32);int32(48);int32(16);int32(0)]')  SignalSizes=str2num('[int32(16);int32(8);int32(16);int32(16)]')  ByteOrders=str2num('[int32(1);int32(1);int32(1);int32(1)]')  DataTypes=str2num('[int32(2);int32(2);int32(2);int32(2)]')  MultiplexTypes=str2num('[int32(1);int32(1);int32(1);int32(1)]')  MultiplexValues=str2num('[double(0);double(0);double(0);double(0)]')  Factors=str2num('[double(1.000000e-01);double(1);double(1.000000e-01);double(1.000000e-01)]')  Offsets=str2num('[double(0);double(-40);double(0);double(0)]')  Minimums=str2num('[double(0);double(-40);double(0);double(0)]')  Maximums=str2num('[double(1000);double(215);double(1000);double(1000)]')  ApplyMinMax=off
      settings: SourceProductName=Simulink Real-Time  SourceProductBaseCode=XP  DataFormat=CANdb specified signals
  Constant : Constant  OutDataTypeStr=uint8
  Constant1 : Constant  OutDataTypeStr=uint8
  Constant4 : Constant  Value=0  OutDataTypeStr=uint8
  Constant5 : Constant  Value=0  OutDataTypeStr=uint8
  Data Store Read : DataStoreRead  DataStoreName=Cnt_DCDC1_1
  Data Store Write : DataStoreWrite  DataStoreName=Cnt_DCDC1_1
  Data Type Conversion{,14..15,17} (4 alike) : DataTypeConversion  OutDataTypeStr=uint8
  Data Type Conversion{1..4} (4 alike) : DataTypeConversion  OutDataTypeStr=single
  Data Type Conversion18 : DataTypeConversion  OutDataTypeStr=uint32
  Data Type Conversion19 : DataTypeConversion  OutDataTypeStr=double
  Message : Outport
  wires:
  Bus Creator1/1 -> Message/1
  Data Type Conversion15/1 -> Bus Creator/3  "Remote"
  Data Type Conversion14/1 -> Bus Creator/2  "Length"
  Data Type Conversion/1 -> Bus Creator/1  "Extended"
  Bus Creator/1 -> CAN Unpack6/1  "CAN_Msg_In"
  Data Type Conversion17/1 -> Bus Creator/4  "Error"
  timestamp/1 -> Data Type Conversion19/1
  Data Type Conversion19/1 -> Bus Creator/6  "Timestamp"
  ID/1 -> Data Type Conversion18/1
  Constant5/1 -> Data Type Conversion17/1
  Constant1/1 -> Data Type Conversion/1
  Data Type Conversion18/1 -> Bus Creator/5  "ID"
  data/1 -> Bus Creator/7  "Data"
  length/1 -> Data Type Conversion14/1
  Constant4/1 -> Data Type Conversion15/1
  CAN Unpack6/1 -> Data Type Conversion1/1
  CAN Unpack6/2 -> Data Type Conversion2/1
  CAN Unpack6/3 -> Data Type Conversion3/1
  CAN Unpack6/4 -> Data Type Conversion4/1
  Data Type Conversion1/1 -> Bus Creator1/1  "DCDC1_InputVolt"
  Data Type Conversion2/1 -> Bus Creator1/2  "DCDC1_ModuleTemp"
  Data Type Conversion3/1 -> Bus Creator1/3  "DCDC1_OutCurr"
  Data Type Conversion4/1 -> Bus Creator1/4  "DCDC1_OutVolt"
  Constant/1 -> Add/2
  Data Store Read/1 -> Add/1
  Add/1 -> Data Store Write/1

== system ZT_VehCtrl_18B_CAN/SigIn/CAN1/DCDC1_2/UNPACK ==
  ID : Inport
  data : Inport  Port=2
  length : Inport  Port=3
  timestamp : Inport  Port=4
  Action Port : ActionPort  ActionType=case
  Add : Sum
  Bus Creator : BusCreator  Inputs=7  OutDataTypeStr=Bus: CAN_MESSAGE_BUS  NonVirtualBus=on
  Bus Creator1 : BusCreator  Inputs=5
  CAN Unpack6 : canmsglib/CAN Unpack  CANdbFile=D:\VCU\VCU_SL_ZhengZhou\ZT2\Module\CAN_DBC\动力CANB_GBK.dbc  MsgList=(none)  MsgName=DCDC1_2  MsgIDType=Extended (29-bit identifier)  MsgIdentifier=402772111  MsgLength=8  SignalInfo=DCDC1_FaultLevel$0$2$1$2$1$0$1$0$0$3$#DCDC1_FaultSt$8$16$1$2$1$0$1$0$0$65535$#DCDC1_HWVersion$48$8$1$2$1$0$1$0$0$255$#DCDC1_SWVersion$56$8$1$2$1$0$1$0$0$255$#DCDC1_WorkSt$2$4$1$2$1$0$1$0$0$15$#  NSignals=5  IDPort=off  TimestampPort=off  ErrorPort=off  RemotePort=off  LengthPort=off  StatusPort=off  StartBits=str2num('[int32(0);int32(8);int32(48);int32(56);int32(2)]')  SignalSizes=str2num('[int32(2);int32(16);int32(8);int32(8);int32(4)]')  ByteOrders=str2num('[int32(1);int32(1);int32(1);int32(1);int32(1)]')  DataTypes=str2num('[int32(2);int32(2);int32(2);int32(2);int32(2)]')  MultiplexTypes=str2num('[int32(1);int32(1);int32(1);int32(1);int32(1)]')  MultiplexValues=str2num('[double(0);double(0);double(0);double(0);double(0)]')  Factors=str2num('[double(1);double(1);double(1);double(1);double(1)]')  Offsets=str2num('[double(0);double(0);double(0);double(0);double(0)]')  Minimums=str2num('[double(0);double(0);double(0);double(0);double(0)]')  Maximums=str2num('[double(3);double(65535);double(255);double(255);double(15)]')  ApplyMinMax=off
      settings: SourceProductName=Simulink Real-Time  SourceProductBaseCode=XP  DataFormat=CANdb specified signals
  Constant : Constant  OutDataTypeStr=uint8
  Constant1 : Constant  OutDataTypeStr=uint8
  Constant4 : Constant  Value=0  OutDataTypeStr=uint8
  Constant5 : Constant  Value=0  OutDataTypeStr=uint8
  Data Store Read : DataStoreRead  DataStoreName=Cnt_DCDC1_2
  Data Store Write : DataStoreWrite  DataStoreName=Cnt_DCDC1_2
  Data Type Conversion{,14..15,17} (4 alike) : DataTypeConversion  OutDataTypeStr=uint8
  Data Type Conversion{1..5} (5 alike) : DataTypeConversion  OutDataTypeStr=single
  Data Type Conversion18 : DataTypeConversion  OutDataTypeStr=uint32
  Data Type Conversion19 : DataTypeConversion  OutDataTypeStr=double
  Message : Outport
  wires:
  Constant4/1 -> Data Type Conversion15/1
  length/1 -> Data Type Conversion14/1
  data/1 -> Bus Creator/7  "Data"
  Data Type Conversion18/1 -> Bus Creator/5  "ID"
  Constant1/1 -> Data Type Conversion/1
  Constant5/1 -> Data Type Conversion17/1
  ID/1 -> Data Type Conversion18/1
  Data Type Conversion19/1 -> Bus Creator/6  "Timestamp"
  timestamp/1 -> Data Type Conversion19/1
  Data Type Conversion17/1 -> Bus Creator/4  "Error"
  Bus Creator/1 -> CAN Unpack6/1  "CAN_Msg_In"
  Data Type Conversion/1 -> Bus Creator/1  "Extended"
  Data Type Conversion14/1 -> Bus Creator/2  "Length"
  Data Type Conversion15/1 -> Bus Creator/3  "Remote"
  Bus Creator1/1 -> Message/1
  CAN Unpack6/1 -> Data Type Conversion1/1
  CAN Unpack6/2 -> Data Type Conversion2/1
  CAN Unpack6/3 -> Data Type Conversion3/1
  CAN Unpack6/4 -> Data Type Conversion4/1
  CAN Unpack6/5 -> Data Type Conversion5/1
  Data Type Conversion1/1 -> Bus Creator1/1  "DCDC1_FaultLevel"
  Data Type Conversion2/1 -> Bus Creator1/2  "DCDC1_FaultSt"
  Data Type Conversion3/1 -> Bus Creator1/3  "DCDC1_HWVersion"
  Data Type Conversion4/1 -> Bus Creator1/4  "DCDC1_SWVersion"
  Data Type Conversion5/1 -> Bus Creator1/5  "DCDC1_WorkSt"
  Add/1 -> Data Store Write/1
  Data Store Read/1 -> Add/1
  Constant/1 -> Add/2

== system ZT_VehCtrl_18B_CAN/SigIn/CAN1/HVC1_LV/UNPACK ==
  ID : Inport
  data : Inport  Port=2
  length : Inport  Port=3
  timestamp : Inport  Port=4
  Action Port : ActionPort  ActionType=case
  Add : Sum
  Bus Creator : BusCreator  Inputs=7  OutDataTypeStr=Bus: CAN_MESSAGE_BUS  NonVirtualBus=on
  Bus Creator1 : BusCreator  Inputs=5
  CAN Unpack6 : canmsglib/CAN Unpack  CANdbFile=D:\VCU\VCU_SL_ZhengZhou\ZT2\模型与接口\CAN_DBC\动力CANB_GBK.dbc  MsgList=(none)  MsgName=HVC1_LV  MsgIDType=Extended (29-bit identifier)  MsgIdentifier=402720161  MsgLength=8  SignalInfo=Batt_Vol$0$8$1$2$1$0$2.000000e-01$0$0$51$#DCDC_OutVol$8$8$1$2$1$0$2.000000e-01$0$0$51$#HVC1_Life$60$4$1$2$1$0$1$0$0$15$#HVC_ChgWakeUpVol$32$8$1$2$1$0$2.000000e-01$0$0$51$#HVC_KL15Vol$24$8$1$2$1$0$2.000000e-01$0$0$51$#  NSignals=5  IDPort=off  TimestampPort=off  ErrorPort=off  RemotePort=off  LengthPort=off  StatusPort=off  StartBits=str2num('[int32(0);int32(8);int32(60);int32(32);int32(24)]')  SignalSizes=str2num('[int32(8);int32(8);int32(4);int32(8);int32(8)]')  ByteOrders=str2num('[int32(1);int32(1);int32(1);int32(1);int32(1)]')  DataTypes=str2num('[int32(2);int32(2);int32(2);int32(2);int32(2)]')  MultiplexTypes=str2num('[int32(1);int32(1);int32(1);int32(1);int32(1)]')  MultiplexValues=str2num('[double(0);double(0);double(0);double(0);double(0)]')  Factors=str2num('[double(2.000000e-01);double(2.000000e-01);double(1);double(2.000000e-01);double(2.000000e-01)]')  Offsets=str2num('[double(0);double(0);double(0);double(0);double(0)]')  Minimums=str2num('[double(0);double(0);double(0);double(0);double(0)]')  Maximums=str2num('[double(51);double(51);double(15);double(51);double(51)]')  ApplyMinMax=off
      settings: SourceProductName=Simulink Real-Time  SourceProductBaseCode=XP  DataFormat=CANdb specified signals
  Constant : Constant  OutDataTypeStr=uint8
  Constant1 : Constant  OutDataTypeStr=uint8
  Constant4 : Constant  Value=0  OutDataTypeStr=uint8
  Constant5 : Constant  Value=0  OutDataTypeStr=uint8
  Data Store Read : DataStoreRead  DataStoreName=Cnt_HVC1
  Data Store Write : DataStoreWrite  DataStoreName=Cnt_HVC1
  Data Type Conversion{,14..15,17} (4 alike) : DataTypeConversion  OutDataTypeStr=uint8
  Data Type Conversion{1..5} (5 alike) : DataTypeConversion  OutDataTypeStr=single
  Data Type Conversion18 : DataTypeConversion  OutDataTypeStr=uint32
  Data Type Conversion19 : DataTypeConversion  OutDataTypeStr=double
  Message : Outport
  wires:
  Constant4/1 -> Data Type Conversion15/1
  length/1 -> Data Type Conversion14/1
  data/1 -> Bus Creator/7  "Data"
  Data Type Conversion18/1 -> Bus Creator/5  "ID"
  Constant1/1 -> Data Type Conversion/1
  Constant5/1 -> Data Type Conversion17/1
  ID/1 -> Data Type Conversion18/1
  Data Type Conversion19/1 -> Bus Creator/6  "Timestamp"
  timestamp/1 -> Data Type Conversion19/1
  Data Type Conversion17/1 -> Bus Creator/4  "Error"
  Bus Creator/1 -> CAN Unpack6/1  "CAN_Msg_In"
  Data Type Conversion/1 -> Bus Creator/1  "Extended"
  Data Type Conversion14/1 -> Bus Creator/2  "Length"
  Data Type Conversion15/1 -> Bus Creator/3  "Remote"
  Bus Creator1/1 -> Message/1
  CAN Unpack6/1 -> Data Type Conversion1/1
  CAN Unpack6/2 -> Data Type Conversion2/1
  CAN Unpack6/3 -> Data Type Conversion3/1
  CAN Unpack6/4 -> Data Type Conversion4/1
  CAN Unpack6/5 -> Data Type Conversion5/1
  Data Type Conversion1/1 -> Bus Creator1/1  "Batt_Vol"
  Data Type Conversion2/1 -> Bus Creator1/2  "DCDC_OutVol"
  Data Type Conversion3/1 -> Bus Creator1/3  "HVC1_Life"
  Data Type Conversion4/1 -> Bus Creator1/4  "HVC_ChgWakeUpVol"
  Data Type Conversion5/1 -> Bus Creator1/5  "HVC_KL15Vol"
  Data Store Read/1 -> Add/1
  Constant/1 -> Add/2
  Add/1 -> Data Store Write/1

== system ZT_VehCtrl_18B_CAN/SigIn/CAN1/HVC3_Temp/UNPACK ==
  ID : Inport
  data : Inport  Port=2
  length : Inport  Port=3
  timestamp : Inport  Port=4
  Action Port : ActionPort  ActionType=case
  Add : Sum
  Bus Creator : BusCreator  Inputs=7  OutDataTypeStr=Bus: CAN_MESSAGE_BUS  NonVirtualBus=on
  Bus Creator1 : BusCreator  Inputs=4
  CAN Unpack6 : canmsglib/CAN Unpack  CANdbFile=D:\VCU\VCU_SL_ZhengZhou\ZT2\模型与接口\CAN_DBC\动力CANB_GBK.dbc  MsgList=(none)  MsgName=HVC3_Temp  MsgIDType=Extended (29-bit identifier)  MsgIdentifier=402851233  MsgLength=8  SignalInfo=HVC3_Life$60$4$1$2$1$0$1$0$0$15$#In_Temp$48$8$1$2$1$0$1$-40$-40$210$#Out_Temp$40$8$1$2$1$0$1$-40$-40$210$#PDU_Temp$0$8$1$2$1$0$1$-40$-40$210$#  NSignals=4  IDPort=off  TimestampPort=off  ErrorPort=off  RemotePort=off  LengthPort=off  StatusPort=off  StartBits=str2num('[int32(60);int32(48);int32(40);int32(0)]')  SignalSizes=str2num('[int32(4);int32(8);int32(8);int32(8)]')  ByteOrders=str2num('[int32(1);int32(1);int32(1);int32(1)]')  DataTypes=str2num('[int32(2);int32(2);int32(2);int32(2)]')  MultiplexTypes=str2num('[int32(1);int32(1);int32(1);int32(1)]')  MultiplexValues=str2num('[double(0);double(0);double(0);double(0)]')  Factors=str2num('[double(1);double(1);double(1);double(1)]')  Offsets=str2num('[double(0);double(-40);double(-40);double(-40)]')  Minimums=str2num('[double(0);double(-40);double(-40);double(-40)]')  Maximums=str2num('[double(15);double(210);double(210);double(210)]')  ApplyMinMax=off
      settings: SourceProductName=Simulink Real-Time  SourceProductBaseCode=XP  DataFormat=CANdb specified signals
  Constant : Constant  OutDataTypeStr=uint8
  Constant1 : Constant  OutDataTypeStr=uint8
  Constant4 : Constant  Value=0  OutDataTypeStr=uint8
  Constant5 : Constant  Value=0  OutDataTypeStr=uint8
  Data Store Read : DataStoreRead  DataStoreName=Cnt_HVC3
  Data Store Write : DataStoreWrite  DataStoreName=Cnt_HVC3
  Data Type Conversion{,14..15,17} (4 alike) : DataTypeConversion  OutDataTypeStr=uint8
  Data Type Conversion{1..4} (4 alike) : DataTypeConversion  OutDataTypeStr=single
  Data Type Conversion18 : DataTypeConversion  OutDataTypeStr=uint32
  Data Type Conversion19 : DataTypeConversion  OutDataTypeStr=double
  Message : Outport
  wires:
  Bus Creator1/1 -> Message/1
  Data Type Conversion15/1 -> Bus Creator/3  "Remote"
  Data Type Conversion14/1 -> Bus Creator/2  "Length"
  Data Type Conversion/1 -> Bus Creator/1  "Extended"
  Bus Creator/1 -> CAN Unpack6/1  "CAN_Msg_In"
  Data Type Conversion17/1 -> Bus Creator/4  "Error"
  timestamp/1 -> Data Type Conversion19/1
  Data Type Conversion19/1 -> Bus Creator/6  "Timestamp"
  ID/1 -> Data Type Conversion18/1
  Constant5/1 -> Data Type Conversion17/1
  Constant1/1 -> Data Type Conversion/1
  Data Type Conversion18/1 -> Bus Creator/5  "ID"
  data/1 -> Bus Creator/7  "Data"
  length/1 -> Data Type Conversion14/1
  Constant4/1 -> Data Type Conversion15/1
  CAN Unpack6/1 -> Data Type Conversion1/1
  CAN Unpack6/2 -> Data Type Conversion2/1
  CAN Unpack6/3 -> Data Type Conversion3/1
  CAN Unpack6/4 -> Data Type Conversion4/1
  Data Type Conversion1/1 -> Bus Creator1/1  "HVC3_Life"
  Data Type Conversion2/1 -> Bus Creator1/2  "In_Temp"
  Data Type Conversion3/1 -> Bus Creator1/3  "Out_Temp"
  Data Type Conversion4/1 -> Bus Creator1/4  "PDU_Temp"
  Add/1 -> Data Store Write/1
  Constant/1 -> Add/2
  Data Store Read/1 -> Add/1
